simulink model "tractor_mu"  (R2022b)
settings: Solver=FixedStepDiscrete  StartTime=0.0  StopTime=20  FixedStep=0.001  RelTol=1e-3
model workspace (MAT data in the model file):
  P : object (value not decoded)
  w_2 : Simulink.Parameter (value not decoded)
undefined symbols (not defined in the file): A, a, B, b, C, D, DiscIntNeverNeededParam, Iz, K, k1, K1, k2, K2, L1, L2, m, magnitude, Phi, Sample_time, Steer_Ratio
libraries: simulink x26, slpidlib x13, Solver_SF x1, dsparch4 x1
(part 3 of 7)

== system tractor_mu/Dugoff轮胎模型/pac2002 ==
  lamda_fl : Inport
  lamda_fr : Inport  Port=2
  lamda_rl : Inport  Port=3
  lamda_rr : Inport  Port=4
  alpha_fl : Inport  Port=5
  alpha_fr : Inport  Port=6
  alpha_rl : Inport  Port=7
  alpha_rr : Inport  Port=8
  Fz_fl : Inport  Port=9
  Fz_rl : Inport  Port=10
  Fz_fr : Inport  Port=11
  Fz_rr : Inport  Port=12
  mu : Inport  Port=13
  Demux : Demux
  Gain{8..11} (4 alike) : Gain  Gain=-1
  fl_dugoff : MATLAB Function  TreatAsAtomicUnit=on
  fr_dugoff : MATLAB Function  TreatAsAtomicUnit=on
  rl_dugoff : MATLAB Function  TreatAsAtomicUnit=on
  rr_dugoff : MATLAB Function  TreatAsAtomicUnit=on
  Fx_fl : Outport
  Fx_fr : Outport  Port=2
  Fx_rl : Outport  Port=3
  Fx_rr : Outport  Port=4
  Fy_fl : Outport  Port=5
  Fy_fr : Outport  Port=6
  Fy_rl : Outport  Port=7
  Fy_rr : Outport  Port=8
  wires:
  alpha_fl/1 -> fl_dugoff/4(alpha)
  Fz_fl/1 -> fl_dugoff/1(Fz)
  alpha_rr/1 -> rr_dugoff/4(alpha)
  Fz_rr/1 -> rr_dugoff/1(Fz)
  [u_fl] -> fl_dugoff/2(u)
  [u_fr] -> fr_dugoff/2(u)
  alpha_fr/1 -> fr_dugoff/4(alpha)
  [u_rl] -> rl_dugoff/2(u)
  [u_rr] -> rr_dugoff/2(u)
  lamda_fr/1 -> Gain11/1
  lamda_rl/1 -> Gain8/1
  lamda_rr/1 -> Gain9/1
  lamda_fl/1 -> Gain10/1
  alpha_rl/1 -> rl_dugoff/4(alpha)
  Gain8/1 -> rl_dugoff/3(lamda)
  Gain9/1 -> rr_dugoff/3(lamda)
  Gain10/1 -> fl_dugoff/3(lamda)
  Gain11/1 -> fr_dugoff/3(lamda)
  mu/1 -> Demux/1
  Demux/1 -> [u_fl]
  Demux/2 -> [u_fr]
  Demux/3 -> [u_rl]
  Demux/4 -> [u_rr]
  Fz_rl/1 -> rl_dugoff/1(Fz)
  Fz_fr/1 -> fr_dugoff/1(Fz)
  fl_dugoff/4(Fy) -> Fy_fl/1
  fl_dugoff/3(Fx) -> Fx_fl/1
  fr_dugoff/4(Fy) -> Fy_fr/1
  fr_dugoff/3(Fx) -> Fx_fr/1
  rl_dugoff/4(Fy) -> Fy_rl/1
  rl_dugoff/3(Fx) -> Fx_rl/1
  rr_dugoff/4(Fy) -> Fy_rr/1
  rr_dugoff/3(Fx) -> Fx_rr/1

== system tractor_mu/PID_Controller//直线循迹/Enabled Subsystem ==
  note: DOB:仿真步长Ts=0.001，时间常数Tao=0.1
      | 如需部署到实车需要根据实车采样频率调整
  yaw_ref : Inport
  yaw : Inport  Port=2
  beta : Inport  Port=3
  omega : Inport  Port=4
  Enable : EnablePort  StatesWhenEnabling=reset
  5500/3000 : slpidlib/PID Controller  Controller=PID  Form=Parallel  TimeDomain=Discrete-time  UseExternalTs=off  SampleTime=-1  IntegratorMethod=Forward Euler  FilterMethod=Forward Euler  ControllerParametersSource=internal  P=5500  I=3500  UseKiTs=off  D=0  N=100  UseFilter=on  TunerSelectOption=Transfer Function Based (PID Tuner App)  InitialConditionSource=internal  InitialConditionForIntegrator=0  InitialConditionForFilter=0  DifferentiatorICPrevScaledInput=0  ExternalReset=none  TrackingMode=off  Kt=1  LimitOutput=off  SatLimitsSource=internal  UpperSaturationLimit=inf  LowerSaturationLimit=-inf  LinearizeAsGain=on  AntiWindupMode=none  Kb=1  LimitIntegrator=off  UpperIntegratorSaturationLimit=inf  LowerIntegratorSaturationLimit=-inf  POutMin=[]  POutMax=[]  IOutMin=[]  IOutMax=[]  DOutMin=[]  DOutMax=[]  NOutMin=[]  NOutMax=[]  SumOutMin=[]  SumOutMax=[]  SaturationOutMin=[]  SaturationOutMax=[]  PParamMin=[]  PParamMax=[]  IParamMin=[]  IParamMax=[]  DParamMin=[]  DParamMax=[]  NParamMin=[]  NParamMax=[]  KbParamMin=[]  KbParamMax=[]  KtParamMin=[]  KtParamMax=[]  KbOutMin=[]  KbOutMax=[]  KtOutMin=[]  KtOutMax=[]  IntegratorOutMin=[]  IntegratorOutMax=[]  FilterOutMin=[]  FilterOutMax=[]  SumI1OutMin=[]  SumI1OutMax=[]  SumI2OutMin=[]  SumI2OutMax=[]  SumI3OutMin=[]  SumI3OutMax=[]  SumI4OutMin=[]  SumI4OutMax=[]  SumDOutMin=[]  SumDOutMax=[]  DifferentiatorOutMin=[]  DifferentiatorOutMax=[]  FilterDiffOutCoefMin=[]  FilterDiffOutCoefMax=[]  ReciprocalOutMin=[]  ReciprocalOutMax=[]  SumDenOutMin=[]  SumDenOutMax=[]  SumNumOutMin=[]  SumNumOutMax=[]  DivideOutMin=[]  DivideOutMax=[]  UdiffTsProdOutMin=[]  UdiffTsProdOutMax=[]  NTsProdOutMin=[]  NTsProdOutMax=[]  UintegralTsProdOutMin=[]  UintegralTsProdOutMax=[]  UngainTsProdOutMin=[]  UngainTsProdOutMax=[]  ClampingZeroOutDataTypeStr=Inherit: Inherit via back propagation  ClampingZeroOutMin=[]  ClampingZeroOutMax=[]  FilterDenConstantOutDataTypeStr=Inherit: Inherit via back propagation  FilterDenConstantOutMin=[]  FilterDenConstantOutMax=[]  PCopyOutDataTypeStr=Inherit: Inherit via back propagation  PCopyOutMin=[]  PCopyOutMax=[]  NCopyOutDataTypeStr=Inherit: Inherit via back propagation  NCopyOutMin=[]  NCopyOutMax=[]  IntegratorContinuousStateAttributes=''  IntegratorStateMustResolveToSignalObject=off  IntegratorRTWStateStorageClass=Auto  FilterContinuousStateAttributes=''  FilterStateMustResolveToSignalObject=off  FilterRTWStateStorageClass=Auto  ParallelPVariant=InternalParameters  IdealPVariant=Disabled  IVariant=InternalParameters  DVariant=InternalParameters  IntegratorVariant=Discrete  SatVariant=Disabled  AWVariant=Passthrough  PCopyVariant=Disabled  TRVariant=Disabled  FdbkBlocksVariant=Forward  IdealPFdbkVariant=Disabled  SatFdbkVariant=Disabled  DerivativeFilterVariant=ForwardEulerFilter  NVariant=InternalParameters  NCopyVariant=Disabled  FilterICVariant=InternalICsFilter  IntegratorICVariant=InternalICs  ExternalResetVariant=Disabled  TRSumVariant=Passthrough  SumFdbkVariant=Disabled  SumVariant=Sum_PID  TsampFilterVariant=InternalTs  TsampNgainVariant=Passthrough  TsampIntegralVariant=Passthrough  ExternalSaturationOutDataTypeStr=Inherit: Same as second input
  Add : Sum  Inputs=+++
  Data Type Conversion : DataTypeConversion  OutDataTypeStr=single  SaturateOnIntegerOverflow=off  RndMeth=Floor
  Data Type Conversion1 : DataTypeConversion  OutDataTypeStr=single  SaturateOnIntegerOverflow=off  RndMeth=Floor
  Discrete Transfer Fcn : DiscreteTransferFcn  Numerator=[1-exp(-0.2)]  Denominator=[1 -exp(-0.2)]
  Gain : Gain  Gain=-1
  Gain1 : Gain  Gain=-K(1)
  Gain2 : Gain  Gain=-K(2)
  Gain3 : Gain  Gain=-K(3)
  Gain4 : Gain  Gain=3
  Gain5 : Gain  Gain=0.5
  Gain6 : Gain  Gain=180/pi
  Izr_dot : simulink/Discrete/Discrete Derivative  gainval=67536  ICPrevScaledInput=0.0  OutMin=[]  OutMax=[]  OutDataType=fixdt(1, 16)  OutScaling=2^-10  DoSatur=off
  Manual Switch : ManualSwitch
  Manual Switch1 : ManualSwitch
  Subtract : Sum  Inputs=+-
  Sum : Sum  Inputs=|+-
  Sum2 : Sum  Inputs=|+-
  Mz : Outport
  wires:
  5500/3000/1 -> Data Type Conversion1/1
  yaw_ref/1 -> Sum/1
  yaw/1 -> Sum/2
  Sum/1 -> Gain/1, Gain6/1
  Sum2/1 -> Manual Switch/2
  Discrete Transfer Fcn/1 -> Gain5/1
  Subtract/1 -> Discrete Transfer Fcn/1
  Gain3/1 -> Add/3  "eyaw"
  Gain1/1 -> Add/1  "beta"
  Izr_dot/1 -> Subtract/1
  omega/1 -> Izr_dot/1, Gain2/1
  Gain2/1 -> Add/2  "omega"
  Add/1 -> Gain4/1
  beta/1 -> Gain1/1
  Gain/1 -> Gain3/1
  Manual Switch/1 -> Manual Switch1/2
  Manual Switch1/1 -> Mz/1
  Gain4/1 -> Subtract/2, Manual Switch/1, Sum2/1
  Data Type Conversion/1 -> Sum2/2  "Mz_DOB"
  Data Type Conversion1/1 -> Manual Switch1/1  "Mz_pid"
  Gain5/1 -> Data Type Conversion/1
  Gain6/1 -> 5500/3000/1

== system tractor_mu/PID_Controller//直线循迹/目标航向角计算 ==
  reset : Inport
  yaw : Inport  Port=2
  omega : Inport  Port=3
  Enable : EnablePort  StatesWhenEnabling=reset
  Abs : Abs  SaturateOnIntegerOverflow=off
  Add : Sum
  Constant : Constant
  Constant1 : Constant  Value=0.001
  Discrete-Time Integrator : DiscreteIntegrator  ExternalReset=rising  SampleTime=-1  ICPrevOutput=DiscIntNeverNeededParam  ICPrevScaledInput=DiscIntNeverNeededParam
  Discrete-Time Integrator1 : DiscreteIntegrator  ExternalReset=rising  SampleTime=-1  ICPrevOutput=DiscIntNeverNeededParam  ICPrevScaledInput=DiscIntNeverNeededParam
  Divide : Product  Inputs=*/
  Divide1 : Product  Inputs=*/
  Product : Product
  Saturation : Saturate  UpperLimit=999999  LowerLimit=0.1
  yaw_r : Outport
  wires:
  Constant/1 -> Divide/1
  omega/1 -> Abs/1
  Abs/1 -> Add/1
  Constant1/1 -> Add/2
  Add/1 -> Divide/2
  Divide/1 -> Discrete-Time Integrator1/1, Product/2
  yaw/1 -> Product/1
  Product/1 -> Discrete-Time Integrator/1
  Discrete-Time Integrator/1 -> Divide1/1
  Discrete-Time Integrator1/1 -> Saturation/1
  Divide1/1 -> yaw_r/1
  Saturation/1 -> Divide1/2
  reset/1 -> Discrete-Time Integrator1/2, Discrete-Time Integrator/2

== system tractor_mu/协同博弈扭矩分配/Subsystem ==
  Tflref : Inport
  Tfrref : Inport  Port=2
  Trlref : Inport  Port=3
  Trrref : Inport  Port=4
  Tflbase : Inport  Port=5
  Tfrbase : Inport  Port=6
  Trlbase : Inport  Port=7
  Trrbase : Inport  Port=8
  alpha : Inport  Port=9
  Constant{,1..3} (4 alike) : Constant
  Product{,1..7} (8 alike) : Product
  Sum{,2,4,6} (4 alike) : Sum  Inputs=|+-
  Sum{1,3,5,7} (4 alike) : Sum  Inputs=|++
  alpha1 : InportShadow  Port=9
  alpha2 : InportShadow  Port=9
  alpha3 : InportShadow  Port=9
  Tfl_sh : Outport
  Tfr_sh : Outport  Port=2
  Trl_sh : Outport  Port=3
  Trr_sh : Outport  Port=4
  wires:
  Tflbase/1 -> Product/1
  Constant/1 -> Sum/1
  alpha/1 -> Sum/2, Product1/2
  Sum/1 -> Product/2
  Product/1 -> Sum1/1
  Product1/1 -> Sum1/2
  Tflref/1 -> Product1/1
  Sum1/1 -> Tfl_sh/1
  Sum3/1 -> Tfr_sh/1
  Tfrref/1 -> Product3/1
  Product3/1 -> Sum3/2
  Product2/1 -> Sum3/1
  Sum2/1 -> Product2/2
  alpha1/1 -> Product3/2, Sum2/2
  Constant1/1 -> Sum2/1
  Tfrbase/1 -> Product2/1
  Trlbase/1 -> Product4/1
  Constant2/1 -> Sum4/1
  alpha2/1 -> Sum4/2, Product5/2
  Sum4/1 -> Product4/2
  Product4/1 -> Sum5/1
  Product5/1 -> Sum5/2
  Trlref/1 -> Product5/1
  Sum5/1 -> Trl_sh/1
  Sum7/1 -> Trr_sh/1
  Trrref/1 -> Product7/1
  Product7/1 -> Sum7/2
  Product6/1 -> Sum7/1
  Sum6/1 -> Product6/2
  alpha3/1 -> Product7/2, Sum6/2
  Constant3/1 -> Sum6/1
  Trrbase/1 -> Product6/1

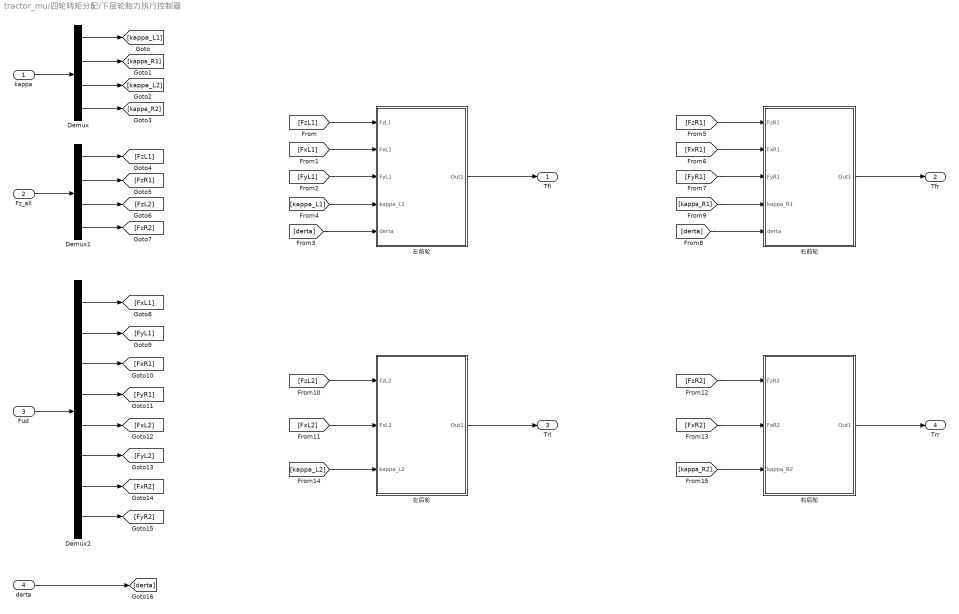
== system tractor_mu/四轮转矩分配/下层轮胎力执行控制器 ==
  kappa : Inport
  Fz_all : Inport  Port=2
  Fud : Inport  Port=3
  derta : Inport  Port=4
  Demux : Demux
  Demux1 : Demux
  Demux2 : Demux  Outputs=8
  右前轮 : Subsystem
  右后轮 : Subsystem
  左前轮 : Subsystem
  左后轮 : Subsystem
  Tfl : Outport
  Tfr : Outport  Port=2
  Trl : Outport  Port=3
  Trr : Outport  Port=4
  wires:
  kappa/1 -> Demux/1
  Demux/1 -> [kappa_L1]
  Demux/2 -> [kappa_R1]
  Demux/3 -> [kappa_L2]
  Demux/4 -> [kappa_R2]
  Fz_all/1 -> Demux1/1
  Demux1/1 -> [FzL1]
  Demux1/2 -> [FzR1]
  Demux1/3 -> [FzL2]
  Demux1/4 -> [FzR2]
  Fud/1 -> Demux2/1
  Demux2/1 -> [FxL1]
  Demux2/2 -> [FyL1]
  Demux2/3 -> [FxR1]
  Demux2/4 -> [FyR1]
  Demux2/6 -> [FyL2]
  Demux2/5 -> [FxL2]
  Demux2/8 -> [FyR2]
  Demux2/7 -> [FxR2]
  derta/1 -> [derta]
  左前轮/1(Out1) -> Tfl/1
  [FzL1] -> 左前轮/1(FzL1)
  [FxL1] -> 左前轮/2(FxL1)
  [FyL1] -> 左前轮/3(FyL1)
  [kappa_L1] -> 左前轮/4(kappa_L1)
  [derta] -> 左前轮/5(derta)
  [derta] -> 右前轮/5(derta)
  [kappa_R1] -> 右前轮/4(kappa_R1)
  [FyR1] -> 右前轮/3(FyR1)
  [FxR1] -> 右前轮/2(FxR1)
  [FzR1] -> 右前轮/1(FzR1)
  右前轮/1(Out1) -> Tfr/1
  [kappa_L2] -> 左后轮/3(kappa_L2)
  [FxL2] -> 左后轮/2(FxL2)
  [FzL2] -> 左后轮/1(FzL2)
  左后轮/1(Out1) -> Trl/1
  右后轮/1(Out1) -> Trr/1
  [FzR2] -> 右后轮/1(FzR2)
  [FxR2] -> 右后轮/2(FxR2)
  [kappa_R2] -> 右后轮/3(kappa_R2)

== system tractor_mu/总驱动力矩制定/DOB补偿 ==
  note: 仿真时间t=0.001
      | 时间常数tao=0.1
  vx : Inport
  T : Inport  Port=2
  Discrete Transfer Fcn : DiscreteTransferFcn  Numerator=[1 1]  Denominator=[201 -199]
  Discrete Derivative : simulink/Discrete/Discrete Derivative  gainval=1.0  ICPrevScaledInput=0.0  OutMin=[]  OutMax=[]  OutDataType=fixdt(1, 16)  OutScaling=2^-10  DoSatur=off
  Sum : Sum  Inputs=|-+
  m*Rf : Gain  Gain=18530*0.834
  低通LPF : DiscreteTransferFcn  Numerator=[1-0.9802]  Denominator=[1 -0.9802]
  Td_hat : Outport
  wires:
  Discrete Derivative/1 -> m*Rf/1
  vx/1 -> 低通LPF/1
  m*Rf/1 -> Sum/1
  T/1 -> Sum/2
  Sum/1 -> Discrete Transfer Fcn/1
  Discrete Transfer Fcn/1 -> Td_hat/1
  低通LPF/1 -> Discrete Derivative/1

== system tractor_mu/总驱动力矩制定/正常工况_高速衰减防抖 ==
  gearD : Inport
  vx : Inport  Port=2
  T0 : Inport  Port=3
  1档 : Switch  Criteria=u2 > Threshold  Threshold=14/3.6  SaturateOnIntegerOverflow=off  InputSameDT=off
  2档 : Switch  Criteria=u2 > Threshold  Threshold=40  SaturateOnIntegerOverflow=off  InputSameDT=off
  Gain14 : Gain  Gain=3.6
  Subsystem1 : Subsystem
  Switch5 : Switch  Criteria=u2 > Threshold  Threshold=1  SaturateOnIntegerOverflow=off  InputSameDT=off
  高速衰减冻结区 : Subsystem
  T : Outport
  wires:
  vx/1 -> 1档/2, Gain14/1
  Gain14/1 -> Subsystem1/1(v), 2档/2, 高速衰减冻结区/1(v)
  T0/1 -> 2档/3, 1档/3
  1档/1 -> Switch5/3
  Subsystem1/1(Out1) -> 2档/1
  高速衰减冻结区/1(Out1) -> 1档/1
  gearD/1 -> Switch5/2
  2档/1 -> Switch5/1
  Switch5/1 -> T/1

== system tractor_mu/牵引效率计算/Subsystem1 ==
  T : Inport
  F_hat : Inport  Port=2
  wij : Inport  Port=3
  Fz : Inport  Port=4
  Add : Sum  Inputs=+++-
  Gain : Gain  Gain=50
  Jw : Gain  Gain=1/356.42
  Product : Product
  Saturation : Saturate  UpperLimit=1  LowerLimit=-1
  Sum : Sum  Inputs=|+-
  边界层厚度 : Gain  Gain=1/1
  Fx_out : Outport
  wires:
  wij/1 -> Sum/1
  Sum/1 -> Gain/1, 边界层厚度/1
  边界层厚度/1 -> Saturation/1
  Saturation/1 -> Product/2  "us"
  T/1 -> Jw/1
  Jw/1 -> Add/1
  Gain/1 -> Add/2
  Product/1 -> Add/3

== system tractor_mu/牵引效率计算/总纵向力估计 ==
  ax : Inport
  theta : Inport  Port=2
  EFsum : Inport  Port=3
  vx : Inport  Port=4
  Fz4 : Inport  Port=5
  Add : Sum  Inputs=---+
  Add1 : Sum  Inputs=++++
  Delay : Delay  DelayLength=1
  Demux : Demux
  Gain1 : Gain  Gain=2.4516
  Gain3 : Gain  Gain=18530*9.8
  Gain5 : Gain  Gain=18530
  Math Function : Math  Operator=magnitude^2
  Saturation : Saturate  UpperLimit=999999999  LowerLimit=0
  Saturation1 : Saturate  UpperLimit=999999999  LowerLimit=0
  Saturation2 : Saturate  UpperLimit=999999999  LowerLimit=0
  Sin1 : Trigonometry
  Sum : Sum  Inputs=|+-
  Switch : Switch  Criteria=u2 > Threshold  Threshold=0.5  SaturateOnIntegerOverflow=off  InputSameDT=off
  滚动阻力系数 : Gain  Gain=0.02
  R_load : Outport
  R_all : Outport  Port=2
  R_g : Outport  Port=3
  R_f : Outport  Port=4
  R_a : Outport  Port=5
  wires:
  ax/1 -> Gain5/1
  theta/1 -> Sin1/1
  Gain1/1 -> R_a/1, Add/2
  Sin1/1 -> Gain3/1
  Gain3/1 -> R_g/1, Add/3
  Add/1 -> Saturation/1
  EFsum/1 -> Sum/1
  Gain5/1 -> Sum/2
  Sum/1 -> Delay/1, Add/4, Saturation1/1
  Fz4/1 -> Demux/1
  Demux/1 -> Add1/1
  Demux/2 -> Add1/2
  Demux/3 -> Add1/3
  Demux/4 -> Add1/4
  Add1/1 -> 滚动阻力系数/1
  滚动阻力系数/1 -> Add/1, R_f/1
  vx/1 -> Switch/2, Math Function/1
  Math Function/1 -> Gain1/1
  Saturation/1 -> R_load/1
  Saturation1/1 -> Switch/1
  Switch/1 -> R_all/1
  Delay/1 -> Saturation2/1
  Saturation2/1 -> Switch/3

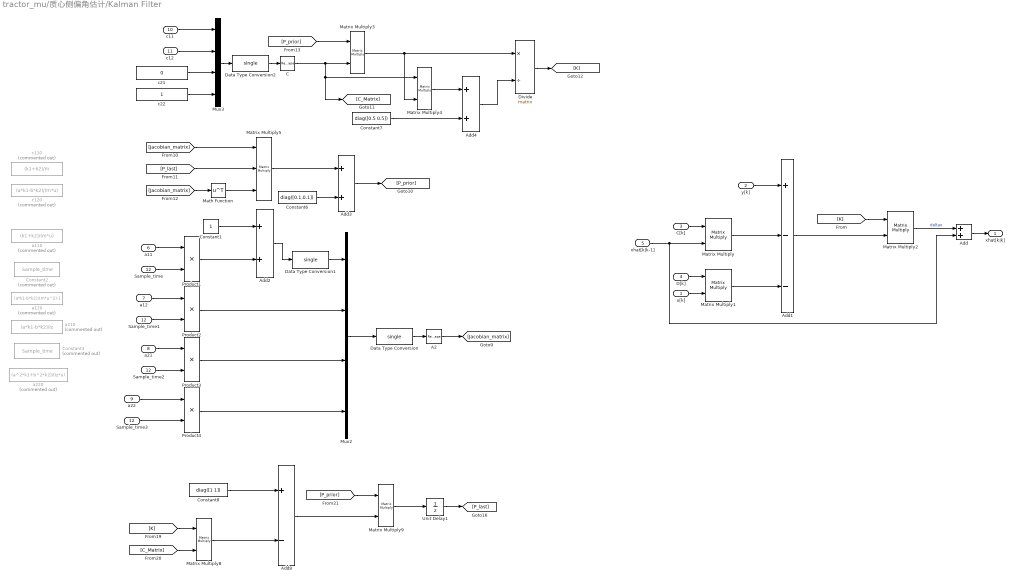
== system tractor_mu/质心侧偏角估计/Kalman Filter ==
  u[k] : Inport
  y[k] : Inport  Port=2
  C[k] : Inport  Port=3
  D[k] : Inport  Port=4
  xhat[k|k-1] : Inport  Port=5
  a11 : Inport  Port=6  OutDataTypeStr=single
  a12 : Inport  Port=7  OutDataTypeStr=single
  a21 : Inport  Port=8  OutDataTypeStr=single
  a22 : Inport  Port=9  OutDataTypeStr=single
  c11 : Inport  Port=10  OutDataTypeStr=single
  c12 : Inport  Port=11  OutDataTypeStr=single
  Sample_time : Inport  Port=12  OutDataTypeStr=single
  A2 : Reshape  OutputDimensionality=Customize  OutputDimensions=[2,2]
  Add{,2..4} (4 alike) : Sum
  Add1 : Sum  Inputs=+--
  Add8 : Sum  Inputs=+-
  C : Reshape  OutputDimensionality=Customize  OutputDimensions=[2,2]
  Constant1 : Constant
  Constant2 : Constant  Commented=on  Value=Sample_time
  Constant3 : Constant  Commented=on  Value=Sample_time
  Constant6 : Constant  Value=diag([0.1,0.1])
  Constant7 : Constant  Value=diag([0.5 0.5])
  Constant8 : Constant  Value=diag([1 1])
  Data Type Conversion : DataTypeConversion  OutDataTypeStr=single  SaturateOnIntegerOverflow=off  RndMeth=Floor
  Data Type Conversion1 : DataTypeConversion  OutDataTypeStr=single  SaturateOnIntegerOverflow=off  RndMeth=Floor
  Data Type Conversion2 : DataTypeConversion  OutDataTypeStr=single  SaturateOnIntegerOverflow=off  RndMeth=Floor
  Divide : Product  Inputs=*/  Multiplication=Matrix(*)
  Math Function : Math  Operator=transpose  SignedPower=on
  Matrix Multiply{,1..4,8..9} (7 alike) : Product  Multiplication=Matrix(*)
  Matrix Multiply5 : Product  Inputs=3  Multiplication=Matrix(*)
  Mux2 : Mux
  Mux3 : Mux
  Product1 : Product
  Product2 : Product
  Product3 : Product  OutDataTypeStr=single
  Product4 : Product  OutDataTypeStr=single
  Sample_time1 : InportShadow  Port=12  OutDataTypeStr=single
  Sample_time2 : InportShadow  Port=12  OutDataTypeStr=single
  Sample_time3 : InportShadow  Port=12  OutDataTypeStr=single
  Unit Delay1 : UnitDelay  SampleTime=-1  HasFrameUpgradeWarning=on
  a110 : Constant  Commented=on  Value=(k1+k2)/(m*u)
  a120 : Constant  Commented=on  Value=(a*k1-b*k2)/(m*u^2)-1
  a210 : Constant  Commented=on  Value=(a*k1-b*k2)/Iz
  a220 : Constant  Commented=on  Value=(a^2*k1+b^2*k2)/(Iz*u)
  c110 : Constant  Commented=on  Value=(k1+k2)/m
  c120 : Constant  Commented=on  Value=(a*k1-b*k2)/(m*u)
  c21 : Constant  Value=0  OutDataTypeStr=single
  c22 : Constant  OutDataTypeStr=single
  xhat[k|k] : Outport
  wires:
  Add/1 -> xhat[k|k]/1
  C[k]/1 -> Matrix Multiply/1
  xhat[k|k-1]/1 -> Matrix Multiply/2, Add/2
  D[k]/1 -> Matrix Multiply1/1
  u[k]/1 -> Matrix Multiply1/2
  y[k]/1 -> Add1/1
  Matrix Multiply/1 -> Add1/2
  Matrix Multiply1/1 -> Add1/3
  Add1/1 -> Matrix Multiply2/2
  Matrix Multiply2/1 -> Add/1  "deltax"
  Add4/1 -> Divide/2
  Matrix Multiply3/1 -> Divide/1, Matrix Multiply4/2
  c21/1 -> Mux3/3
  Matrix Multiply4/1 -> Add4/1
  c22/1 -> Mux3/4
  Mux3/1 -> Data Type Conversion2/1
  Constant7/1 -> Add4/2
  c11/1 -> Mux3/1
  [P_prior] -> Matrix Multiply3/1
  C/1 -> Matrix Multiply4/1, [C_Matrix], Matrix Multiply3/2
  Divide/1 -> [K]
  [P_last] -> Matrix Multiply5/2
  Matrix Multiply5/1 -> Add3/1
  [Jacobian_matrix] -> Math Function/1
  Math Function/1 -> Matrix Multiply5/3
  Add3/1 -> [P_prior]
  [Jacobian_matrix] -> Matrix Multiply5/1
  Constant6/1 -> Add3/2
  Sample_time2/1 -> Product3/2
  Sample_time3/1 -> Product4/2
  a12/1 -> Product2/1
  A2/1 -> [Jacobian_matrix]
  Add2/1 -> Data Type Conversion1/1
  Product1/1 -> Add2/2
  Sample_time1/1 -> Product2/2
  a22/1 -> Product4/1
  Mux2/1 -> Data Type Conversion/1
  a21/1 -> Product3/1
  Constant1/1 -> Add2/1
  [K] -> Matrix Multiply2/1
  Matrix Multiply8/1 -> Add8/2
  Constant8/1 -> Add8/1
  Unit Delay1/1 -> [P_last]
  [P_prior] -> Matrix Multiply9/1
  Add8/1 -> Matrix Multiply9/2
  Matrix Multiply9/1 -> Unit Delay1/1
  [K] -> Matrix Multiply8/1
  [C_Matrix] -> Matrix Multiply8/2
  a11/1 -> Product1/1
  c12/1 -> Mux3/2
  Sample_time/1 -> Product1/2
  Product2/1 -> Mux2/2
  Product3/1 -> Mux2/3
  Product4/1 -> Mux2/4
  Data Type Conversion/1 -> A2/1
  Data Type Conversion1/1 -> Mux2/1
  Data Type Conversion2/1 -> C/1

== system tractor_mu/质心侧偏角估计/Observer ==
  note: A*xhat+B*u+L*(yMeas-yHat)
      | or
      | A*xhat+B*u
  u[k] : Inport
  y[k] : Inport  Port=2
  A[k] : Inport  Port=3
  B[k] : Inport  Port=4
  C[k] : Inport  Port=5
  D[k] : Inport  Port=6
  L[k] : Inport  Port=7
  xhat[k|k-1] : Inport  Port=8
  Add : Sum  Inputs=+++
  Matrix Multiply : Product  Multiplication=Matrix(*)
  Matrix Multiply1 : Product  Multiplication=Matrix(*)
  Reshape : Reshape
  Subsystem : Subsystem
  x[k+1|k] : Outport
  wires:
  B[k]/1 -> Matrix Multiply/1
  u[k]/1 -> Subsystem/6(u[k]), Matrix Multiply/2
  A[k]/1 -> Matrix Multiply1/1
  xhat[k|k-1]/1 -> Matrix Multiply1/2, Subsystem/4(xhat[k|k-1])
  L[k]/1 -> Subsystem/1(L[k])
  y[k]/1 -> Subsystem/2(y[k])
  C[k]/1 -> Subsystem/3(C[k])
  D[k]/1 -> Subsystem/5(D[k])
  Matrix Multiply/1 -> Add/1
  Matrix Multiply1/1 -> Add/2
  Subsystem/1(L*(y[k]-yhat[k|k-1])) -> Add/3
  Add/1 -> Reshape/1
  Reshape/1 -> x[k+1|k]/1

== system tractor_mu/质心侧偏角滑模观测器估计/Subsystem ==
  Avz_Carsim : Inport
  vx : Inport  Port=2
  delta_f : Inport  Port=3
  Atan : Trigonometry  Operator=atan
  Constant : Constant  Value=0.1
  Divide : Product  Inputs=*/
  Gain1 : Gain  Gain=L1
  Gain2 : Gain  Gain=L2
  MATLAB Function : MATLAB Function  TreatAsAtomicUnit=on  SystemSampleTime=0.005
  Scope1 : Scope
  Scope2 : Scope
  Subsystem : Subsystem
  Sum : Sum  Inputs=|+-
  Sum1 : Sum  Inputs=|++
  Sum2 : Sum  Inputs=|++
  Switch : Switch  Criteria=u2 > Threshold  Threshold=0.1  SaturateOnIntegerOverflow=off  InputSameDT=off
  gamma_hat : DiscreteIntegrator  SampleTime=-1  ICPrevOutput=DiscIntNeverNeededParam  ICPrevScaledInput=DiscIntNeverNeededParam
  vy_hat : DiscreteIntegrator  SampleTime=-1  ICPrevOutput=DiscIntNeverNeededParam  ICPrevScaledInput=DiscIntNeverNeededParam
  beta_est : Outport
  gamma_est : Outport  Port=2
  vy_hat_output : Outport  Port=3
  wires:
  Avz_Carsim/1 -> Sum/1
  Sum/1 -> Subsystem/1(error)
  MATLAB Function/1(d_vy_model) -> Sum1/2
  gamma_hat/1 -> Scope1/1, MATLAB Function/4(gamma_hat), gamma_est/1, Sum/2
  vx/1 -> Scope2/1, Switch/1, Switch/2
  Constant/1 -> Switch/3
  vy_hat/1 -> vy_hat_output/1, Divide/1, MATLAB Function/3(vy_hat)
  Switch/1 -> Divide/2, MATLAB Function/1(vx)
  Subsystem/1(v_STA) -> Gain2/1, Gain1/1
  delta_f/1 -> MATLAB Function/2(delta_f)
  Divide/1 -> Atan/1
  Gain1/1 -> Sum1/1
  Gain2/1 -> Sum2/1
  MATLAB Function/2(d_gamma_model) -> Sum2/2
  Atan/1 -> beta_est/1
  Sum1/1 -> vy_hat/1
  Sum2/1 -> gamma_hat/1

== system tractor_mu/质心侧偏角滑模观测器估计/Subsystem1 ==
  Avz_Carsim : Inport
  vx : Inport  Port=2
  delta_f : Inport  Port=3
  Atan : Trigonometry  Operator=atan
  Constant : Constant  Value=0.1
  Divide : Product  Inputs=*/
  Gain : Gain  Gain=1/Phi
  Gain1 : Gain  Gain=L1
  Gain2 : Gain  Gain=L2
  MATLAB Function : MATLAB Function  TreatAsAtomicUnit=on  SystemSampleTime=0.005
  Saturation : Saturate  UpperLimit=1  LowerLimit=-1
  Scope1 : Scope
  Scope2 : Scope
  Sum : Sum  Inputs=|+-
  Sum1 : Sum  Inputs=|++
  Sum2 : Sum  Inputs=|++
  Switch : Switch  Criteria=u2 > Threshold  Threshold=0.1  SaturateOnIntegerOverflow=off  InputSameDT=off
  gamma_hat : Integrator
  vy_hat : Integrator
  beta_est : Outport
  gamma_est : Outport  Port=2
  vy_hat_output : Outport  Port=3
  wires:
  Gain/1 -> Saturation/1
  Avz_Carsim/1 -> Sum/1
  Sum/1 -> Gain/1
  MATLAB Function/1(d_vy_model) -> Sum1/2
  gamma_hat/1 -> Scope1/1, MATLAB Function/4(gamma_hat), gamma_est/1, Sum/2
  vx/1 -> Scope2/1, Switch/1, Switch/2
  Constant/1 -> Switch/3
  vy_hat/1 -> vy_hat_output/1, Divide/1, MATLAB Function/3(vy_hat)
  Switch/1 -> Divide/2, MATLAB Function/1(vx)
  Saturation/1 -> Gain2/1, Gain1/1
  delta_f/1 -> MATLAB Function/2(delta_f)
  Divide/1 -> Atan/1
  Gain1/1 -> Sum1/1
  Gain2/1 -> Sum2/1
  MATLAB Function/2(d_gamma_model) -> Sum2/2
  Atan/1 -> beta_est/1
  Sum1/1 -> vy_hat/1
  Sum2/1 -> gamma_hat/1

== system tractor_mu/驱动防滑模块/Subsystem ==
  lamda1 : Inport
  p : Inport  Port=2
  i : Inport  Port=3
  b : Inport  Port=4
  Constant : Constant  Value=0.2
  PID Controller : slpidlib/PID Controller  Controller=PI  Form=Parallel  TimeDomain=Discrete-time  UseExternalTs=off  SampleTime=-1  IntegratorMethod=Forward Euler  FilterMethod=Forward Euler  ControllerParametersSource=external  P=5000  I=3000  UseKiTs=off  D=0  N=100  UseFilter=on  TunerSelectOption=Transfer Function Based (PID Tuner App)  InitialConditionSource=internal  InitialConditionForIntegrator=0  InitialConditionForFilter=0  DifferentiatorICPrevScaledInput=0  ExternalReset=none  TrackingMode=off  Kt=1  LimitOutput=on  SatLimitsSource=internal  UpperSaturationLimit=0  LowerSaturationLimit=-30000  LinearizeAsGain=on  AntiWindupMode=clamping  Kb=1  LimitIntegrator=off  UpperIntegratorSaturationLimit=inf  LowerIntegratorSaturationLimit=-inf  POutMin=[]  POutMax=[]  IOutMin=[]  IOutMax=[]  DOutMin=[]  DOutMax=[]  NOutMin=[]  NOutMax=[]  SumOutMin=[]  SumOutMax=[]  SaturationOutMin=[]  SaturationOutMax=[]  PParamMin=[]  PParamMax=[]  IParamMin=[]  IParamMax=[]  DParamMin=[]  DParamMax=[]  NParamMin=[]  NParamMax=[]  KbParamMin=[]  KbParamMax=[]  KtParamMin=[]  KtParamMax=[]  KbOutMin=[]  KbOutMax=[]  KtOutMin=[]  KtOutMax=[]  IntegratorOutMin=[]  IntegratorOutMax=[]  FilterOutMin=[]  FilterOutMax=[]  SumI1OutMin=[]  SumI1OutMax=[]  SumI2OutMin=[]  SumI2OutMax=[]  SumI3OutMin=[]  SumI3OutMax=[]  SumI4OutMin=[]  SumI4OutMax=[]  SumDOutMin=[]  SumDOutMax=[]  DifferentiatorOutMin=[]  DifferentiatorOutMax=[]  FilterDiffOutCoefMin=[]  FilterDiffOutCoefMax=[]  ReciprocalOutMin=[]  ReciprocalOutMax=[]  SumDenOutMin=[]  SumDenOutMax=[]  SumNumOutMin=[]  SumNumOutMax=[]  DivideOutMin=[]  DivideOutMax=[]  UdiffTsProdOutMin=[]  UdiffTsProdOutMax=[]  NTsProdOutMin=[]  NTsProdOutMax=[]  UintegralTsProdOutMin=[]  UintegralTsProdOutMax=[]  UngainTsProdOutMin=[]  UngainTsProdOutMax=[]  ClampingZeroOutDataTypeStr=Inherit: Inherit via back propagation  ClampingZeroOutMin=[]  ClampingZeroOutMax=[]  FilterDenConstantOutDataTypeStr=Inherit: Inherit via back propagation  FilterDenConstantOutMin=[]  FilterDenConstantOutMax=[]  PCopyOutDataTypeStr=Inherit: Inherit via back propagation  PCopyOutMin=[]  PCopyOutMax=[]  NCopyOutDataTypeStr=Inherit: Inherit via back propagation  NCopyOutMin=[]  NCopyOutMax=[]  IntegratorContinuousStateAttributes=''  IntegratorStateMustResolveToSignalObject=off  IntegratorRTWStateStorageClass=Auto  FilterContinuousStateAttributes=''  FilterStateMustResolveToSignalObject=off  FilterRTWStateStorageClass=Auto  ParallelPVariant=ExternalParameters  IdealPVariant=Disabled  IVariant=ExternalParameters  DVariant=Disabled  IntegratorVariant=Discrete  SatVariant=Enabled  AWVariant=DiscClampingParallel  PCopyVariant=Disabled  TRVariant=Disabled  FdbkBlocksVariant=Forward  IdealPFdbkVariant=Disabled  SatFdbkVariant=Disabled  DerivativeFilterVariant=Disabled  NVariant=Disabled  NCopyVariant=Disabled_SignalSpec  FilterICVariant=Disabled  IntegratorICVariant=InternalICs  ExternalResetVariant=Disabled  TRSumVariant=Passthrough  SumFdbkVariant=Disabled  SumVariant=Sum_PI  TsampFilterVariant=InternalTs  TsampNgainVariant=Passthrough  TsampIntegralVariant=Passthrough  ExternalSaturationOutDataTypeStr=Inherit: Same as second input
  Saturation : Saturate  UpperLimit=30000  LowerLimit=-30000
  Sum4 : Sum  Inputs=|+-
  dT1 : Outport
  wires:
  Sum4/1 -> PID Controller/1
  lamda1/1 -> Sum4/2
  PID Controller/1 -> Saturation/1  "dT1"
  p/1 -> PID Controller/2
  i/1 -> PID Controller/3
  Constant/1 -> Sum4/1
  Saturation/1 -> dT1/1

== system tractor_mu/驱动防滑模块/Subsystem1 ==
  lamda2 : Inport
  p : Inport  Port=2
  i : Inport  Port=3
  b : Inport  Port=4
  Constant : Constant  Value=0.2
  PID Controller : slpidlib/PID Controller  Controller=PI  Form=Parallel  TimeDomain=Discrete-time  UseExternalTs=off  SampleTime=-1  IntegratorMethod=Forward Euler  FilterMethod=Forward Euler  ControllerParametersSource=external  P=5000  I=3000  UseKiTs=off  D=0  N=100  UseFilter=on  TunerSelectOption=Transfer Function Based (PID Tuner App)  InitialConditionSource=internal  InitialConditionForIntegrator=0  InitialConditionForFilter=0  DifferentiatorICPrevScaledInput=0  ExternalReset=none  TrackingMode=off  Kt=1  LimitOutput=on  SatLimitsSource=internal  UpperSaturationLimit=0  LowerSaturationLimit=-30000  LinearizeAsGain=on  AntiWindupMode=clamping  Kb=1  LimitIntegrator=off  UpperIntegratorSaturationLimit=inf  LowerIntegratorSaturationLimit=-inf  POutMin=[]  POutMax=[]  IOutMin=[]  IOutMax=[]  DOutMin=[]  DOutMax=[]  NOutMin=[]  NOutMax=[]  SumOutMin=[]  SumOutMax=[]  SaturationOutMin=[]  SaturationOutMax=[]  PParamMin=[]  PParamMax=[]  IParamMin=[]  IParamMax=[]  DParamMin=[]  DParamMax=[]  NParamMin=[]  NParamMax=[]  KbParamMin=[]  KbParamMax=[]  KtParamMin=[]  KtParamMax=[]  KbOutMin=[]  KbOutMax=[]  KtOutMin=[]  KtOutMax=[]  IntegratorOutMin=[]  IntegratorOutMax=[]  FilterOutMin=[]  FilterOutMax=[]  SumI1OutMin=[]  SumI1OutMax=[]  SumI2OutMin=[]  SumI2OutMax=[]  SumI3OutMin=[]  SumI3OutMax=[]  SumI4OutMin=[]  SumI4OutMax=[]  SumDOutMin=[]  SumDOutMax=[]  DifferentiatorOutMin=[]  DifferentiatorOutMax=[]  FilterDiffOutCoefMin=[]  FilterDiffOutCoefMax=[]  ReciprocalOutMin=[]  ReciprocalOutMax=[]  SumDenOutMin=[]  SumDenOutMax=[]  SumNumOutMin=[]  SumNumOutMax=[]  DivideOutMin=[]  DivideOutMax=[]  UdiffTsProdOutMin=[]  UdiffTsProdOutMax=[]  NTsProdOutMin=[]  NTsProdOutMax=[]  UintegralTsProdOutMin=[]  UintegralTsProdOutMax=[]  UngainTsProdOutMin=[]  UngainTsProdOutMax=[]  ClampingZeroOutDataTypeStr=Inherit: Inherit via back propagation  ClampingZeroOutMin=[]  ClampingZeroOutMax=[]  FilterDenConstantOutDataTypeStr=Inherit: Inherit via back propagation  FilterDenConstantOutMin=[]  FilterDenConstantOutMax=[]  PCopyOutDataTypeStr=Inherit: Inherit via back propagation  PCopyOutMin=[]  PCopyOutMax=[]  NCopyOutDataTypeStr=Inherit: Inherit via back propagation  NCopyOutMin=[]  NCopyOutMax=[]  IntegratorContinuousStateAttributes=''  IntegratorStateMustResolveToSignalObject=off  IntegratorRTWStateStorageClass=Auto  FilterContinuousStateAttributes=''  FilterStateMustResolveToSignalObject=off  FilterRTWStateStorageClass=Auto  ParallelPVariant=ExternalParameters  IdealPVariant=Disabled  IVariant=ExternalParameters  DVariant=Disabled  IntegratorVariant=Discrete  SatVariant=Enabled  AWVariant=DiscClampingParallel  PCopyVariant=Disabled  TRVariant=Disabled  FdbkBlocksVariant=Forward  IdealPFdbkVariant=Disabled  SatFdbkVariant=Disabled  DerivativeFilterVariant=Disabled  NVariant=Disabled  NCopyVariant=Disabled_SignalSpec  FilterICVariant=Disabled  IntegratorICVariant=InternalICs  ExternalResetVariant=Disabled  TRSumVariant=Passthrough  SumFdbkVariant=Disabled  SumVariant=Sum_PI  TsampFilterVariant=InternalTs  TsampNgainVariant=Passthrough  TsampIntegralVariant=Passthrough  ExternalSaturationOutDataTypeStr=Inherit: Same as second input
  Saturation : Saturate  UpperLimit=30000  LowerLimit=-99999
  Sum4 : Sum  Inputs=|+-
  dT1 : Outport
  wires:
  i/1 -> PID Controller/3
  p/1 -> PID Controller/2
  PID Controller/1 -> Saturation/1  "dT1"
  lamda2/1 -> Sum4/2
  Sum4/1 -> PID Controller/1
  Saturation/1 -> dT1/1
  Constant/1 -> Sum4/1

== system tractor_mu/驱动防滑模块/Subsystem2 ==
  lamda3 : Inport
  p : Inport  Port=2
  i : Inport  Port=3
  b : Inport  Port=4
  Constant : Constant  Value=0.2
  PID Controller : slpidlib/PID Controller  Controller=PI  Form=Parallel  TimeDomain=Discrete-time  UseExternalTs=off  SampleTime=-1  IntegratorMethod=Forward Euler  FilterMethod=Forward Euler  ControllerParametersSource=external  P=5000  I=3000  UseKiTs=off  D=0  N=100  UseFilter=on  TunerSelectOption=Transfer Function Based (PID Tuner App)  InitialConditionSource=internal  InitialConditionForIntegrator=0  InitialConditionForFilter=0  DifferentiatorICPrevScaledInput=0  ExternalReset=none  TrackingMode=off  Kt=1  LimitOutput=on  SatLimitsSource=internal  UpperSaturationLimit=0  LowerSaturationLimit=-50000  LinearizeAsGain=on  AntiWindupMode=clamping  Kb=1  LimitIntegrator=off  UpperIntegratorSaturationLimit=inf  LowerIntegratorSaturationLimit=-inf  POutMin=[]  POutMax=[]  IOutMin=[]  IOutMax=[]  DOutMin=[]  DOutMax=[]  NOutMin=[]  NOutMax=[]  SumOutMin=[]  SumOutMax=[]  SaturationOutMin=[]  SaturationOutMax=[]  PParamMin=[]  PParamMax=[]  IParamMin=[]  IParamMax=[]  DParamMin=[]  DParamMax=[]  NParamMin=[]  NParamMax=[]  KbParamMin=[]  KbParamMax=[]  KtParamMin=[]  KtParamMax=[]  KbOutMin=[]  KbOutMax=[]  KtOutMin=[]  KtOutMax=[]  IntegratorOutMin=[]  IntegratorOutMax=[]  FilterOutMin=[]  FilterOutMax=[]  SumI1OutMin=[]  SumI1OutMax=[]  SumI2OutMin=[]  SumI2OutMax=[]  SumI3OutMin=[]  SumI3OutMax=[]  SumI4OutMin=[]  SumI4OutMax=[]  SumDOutMin=[]  SumDOutMax=[]  DifferentiatorOutMin=[]  DifferentiatorOutMax=[]  FilterDiffOutCoefMin=[]  FilterDiffOutCoefMax=[]  ReciprocalOutMin=[]  ReciprocalOutMax=[]  SumDenOutMin=[]  SumDenOutMax=[]  SumNumOutMin=[]  SumNumOutMax=[]  DivideOutMin=[]  DivideOutMax=[]  UdiffTsProdOutMin=[]  UdiffTsProdOutMax=[]  NTsProdOutMin=[]  NTsProdOutMax=[]  UintegralTsProdOutMin=[]  UintegralTsProdOutMax=[]  UngainTsProdOutMin=[]  UngainTsProdOutMax=[]  ClampingZeroOutDataTypeStr=Inherit: Inherit via back propagation  ClampingZeroOutMin=[]  ClampingZeroOutMax=[]  FilterDenConstantOutDataTypeStr=Inherit: Inherit via back propagation  FilterDenConstantOutMin=[]  FilterDenConstantOutMax=[]  PCopyOutDataTypeStr=Inherit: Inherit via back propagation  PCopyOutMin=[]  PCopyOutMax=[]  NCopyOutDataTypeStr=Inherit: Inherit via back propagation  NCopyOutMin=[]  NCopyOutMax=[]  IntegratorContinuousStateAttributes=''  IntegratorStateMustResolveToSignalObject=off  IntegratorRTWStateStorageClass=Auto  FilterContinuousStateAttributes=''  FilterStateMustResolveToSignalObject=off  FilterRTWStateStorageClass=Auto  ParallelPVariant=ExternalParameters  IdealPVariant=Disabled  IVariant=ExternalParameters  DVariant=Disabled  IntegratorVariant=Discrete  SatVariant=Enabled  AWVariant=DiscClampingParallel  PCopyVariant=Disabled  TRVariant=Disabled  FdbkBlocksVariant=Forward  IdealPFdbkVariant=Disabled  SatFdbkVariant=Disabled  DerivativeFilterVariant=Disabled  NVariant=Disabled  NCopyVariant=Disabled_SignalSpec  FilterICVariant=Disabled  IntegratorICVariant=InternalICs  ExternalResetVariant=Disabled  TRSumVariant=Passthrough  SumFdbkVariant=Disabled  SumVariant=Sum_PI  TsampFilterVariant=InternalTs  TsampNgainVariant=Passthrough  TsampIntegralVariant=Passthrough  ExternalSaturationOutDataTypeStr=Inherit: Same as second input
  Saturation : Saturate  UpperLimit=30000  LowerLimit=-99999
  Sum4 : Sum  Inputs=|+-
  dT1 : Outport
  wires:
  Sum4/1 -> PID Controller/1
  lamda3/1 -> Sum4/2
  PID Controller/1 -> Saturation/1  "dT1"
  p/1 -> PID Controller/2
  i/1 -> PID Controller/3
  Saturation/1 -> dT1/1
  Constant/1 -> Sum4/1

== system tractor_mu/驱动防滑模块/Subsystem3 ==
  lamda4 : Inport
  p : Inport  Port=2
  i : Inport  Port=3
  b : Inport  Port=4
  Constant : Constant  Value=0.2
  PID Controller : slpidlib/PID Controller  Controller=PI  Form=Parallel  TimeDomain=Discrete-time  UseExternalTs=off  SampleTime=-1  IntegratorMethod=Forward Euler  FilterMethod=Forward Euler  ControllerParametersSource=external  P=5000  I=3000  UseKiTs=off  D=0  N=100  UseFilter=on  TunerSelectOption=Transfer Function Based (PID Tuner App)  InitialConditionSource=internal  InitialConditionForIntegrator=0  InitialConditionForFilter=0  DifferentiatorICPrevScaledInput=0  ExternalReset=none  TrackingMode=off  Kt=1  LimitOutput=on  SatLimitsSource=internal  UpperSaturationLimit=0  LowerSaturationLimit=-50000  LinearizeAsGain=on  AntiWindupMode=clamping  Kb=1  LimitIntegrator=off  UpperIntegratorSaturationLimit=inf  LowerIntegratorSaturationLimit=-inf  POutMin=[]  POutMax=[]  IOutMin=[]  IOutMax=[]  DOutMin=[]  DOutMax=[]  NOutMin=[]  NOutMax=[]  SumOutMin=[]  SumOutMax=[]  SaturationOutMin=[]  SaturationOutMax=[]  PParamMin=[]  PParamMax=[]  IParamMin=[]  IParamMax=[]  DParamMin=[]  DParamMax=[]  NParamMin=[]  NParamMax=[]  KbParamMin=[]  KbParamMax=[]  KtParamMin=[]  KtParamMax=[]  KbOutMin=[]  KbOutMax=[]  KtOutMin=[]  KtOutMax=[]  IntegratorOutMin=[]  IntegratorOutMax=[]  FilterOutMin=[]  FilterOutMax=[]  SumI1OutMin=[]  SumI1OutMax=[]  SumI2OutMin=[]  SumI2OutMax=[]  SumI3OutMin=[]  SumI3OutMax=[]  SumI4OutMin=[]  SumI4OutMax=[]  SumDOutMin=[]  SumDOutMax=[]  DifferentiatorOutMin=[]  DifferentiatorOutMax=[]  FilterDiffOutCoefMin=[]  FilterDiffOutCoefMax=[]  ReciprocalOutMin=[]  ReciprocalOutMax=[]  SumDenOutMin=[]  SumDenOutMax=[]  SumNumOutMin=[]  SumNumOutMax=[]  DivideOutMin=[]  DivideOutMax=[]  UdiffTsProdOutMin=[]  UdiffTsProdOutMax=[]  NTsProdOutMin=[]  NTsProdOutMax=[]  UintegralTsProdOutMin=[]  UintegralTsProdOutMax=[]  UngainTsProdOutMin=[]  UngainTsProdOutMax=[]  ClampingZeroOutDataTypeStr=Inherit: Inherit via back propagation  ClampingZeroOutMin=[]  ClampingZeroOutMax=[]  FilterDenConstantOutDataTypeStr=Inherit: Inherit via back propagation  FilterDenConstantOutMin=[]  FilterDenConstantOutMax=[]  PCopyOutDataTypeStr=Inherit: Inherit via back propagation  PCopyOutMin=[]  PCopyOutMax=[]  NCopyOutDataTypeStr=Inherit: Inherit via back propagation  NCopyOutMin=[]  NCopyOutMax=[]  IntegratorContinuousStateAttributes=''  IntegratorStateMustResolveToSignalObject=off  IntegratorRTWStateStorageClass=Auto  FilterContinuousStateAttributes=''  FilterStateMustResolveToSignalObject=off  FilterRTWStateStorageClass=Auto  ParallelPVariant=ExternalParameters  IdealPVariant=Disabled  IVariant=ExternalParameters  DVariant=Disabled  IntegratorVariant=Discrete  SatVariant=Enabled  AWVariant=DiscClampingParallel  PCopyVariant=Disabled  TRVariant=Disabled  FdbkBlocksVariant=Forward  IdealPFdbkVariant=Disabled  SatFdbkVariant=Disabled  DerivativeFilterVariant=Disabled  NVariant=Disabled  NCopyVariant=Disabled_SignalSpec  FilterICVariant=Disabled  IntegratorICVariant=InternalICs  ExternalResetVariant=Disabled  TRSumVariant=Passthrough  SumFdbkVariant=Disabled  SumVariant=Sum_PI  TsampFilterVariant=InternalTs  TsampNgainVariant=Passthrough  TsampIntegralVariant=Passthrough  ExternalSaturationOutDataTypeStr=Inherit: Same as second input
  Saturation : Saturate  UpperLimit=30000  LowerLimit=-99999
  Sum4 : Sum  Inputs=|+-
  dT1 : Outport
  wires:
  i/1 -> PID Controller/3
  p/1 -> PID Controller/2
  PID Controller/1 -> Saturation/1  "dT1"
  lamda4/1 -> Sum4/2
  Sum4/1 -> PID Controller/1
  Saturation/1 -> dT1/1
  Constant/1 -> Sum4/1

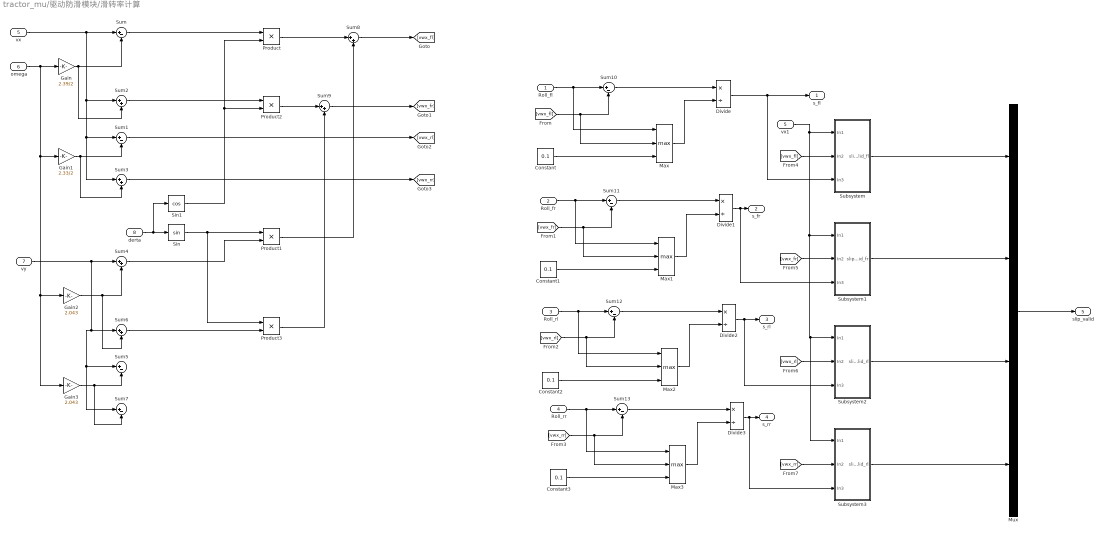
== system tractor_mu/驱动防滑模块/滑转率计算 ==
  Roll_fl : Inport
  Roll_fr : Inport  Port=2
  Roll_rl : Inport  Port=3
  Roll_rr : Inport  Port=4
  vx : Inport  Port=5
  omega : Inport  Port=6
  vy : Inport  Port=7
  derta : Inport  Port=8
  Constant{,1..3} (4 alike) : Constant  Value=0.1
  Divide{,1..3} (4 alike) : Product  Inputs=*/
  Gain : Gain  Gain=2.39/2
  Gain1 : Gain  Gain=2.33/2
  Gain2 : Gain  Gain=2.043
  Gain3 : Gain  Gain=2.043
  Max{,1..3} (4 alike) : MinMax  Function=max  Inputs=3
  Mux : Mux
  Product{,1..3} (4 alike) : Product
  Sin : Trigonometry
  Sin1 : Trigonometry  Operator=cos
  Subsystem : Subsystem
  Subsystem1 : Subsystem
  Subsystem2 : Subsystem
  Subsystem3 : Subsystem
  Sum{,1,5,7,10..13} (8 alike) : Sum  Inputs=|+-
  Sum{2..4,6,8..9} (6 alike) : Sum  Inputs=|++
  vx1 : InportShadow  Port=5
  s_fl : Outport
  s_fr : Outport  Port=2
  s_rl : Outport  Port=3
  s_rr : Outport  Port=4
  slip_valid : Outport  Port=5
  wires:
  vx/1 -> Sum3/1, Sum1/1, Sum2/1, Sum/1
  Gain/1 -> Sum2/2, Sum/2
  Gain1/1 -> Sum3/2, Sum1/2
  Gain3/1 -> Sum5/2, Sum7/2
  Gain2/1 -> Sum4/2, Sum6/2
  omega/1 -> Gain3/1, Gain2/1, Gain1/1, Gain/1
  vy/1 -> Sum4/1, Sum5/1, Sum7/1, Sum6/1
  derta/1 -> Sin1/1, Sin/1
  Sum/1 -> Product/1
  Sin1/1 -> Product2/2, Product/2
  Product/1 -> Sum8/1
  Sin/1 -> Product3/1, Product1/1
  Sum4/1 -> Product1/2
  Product1/1 -> Sum8/2
  Sum8/1 -> [vwx_fl]
  Sum2/1 -> Product2/1
  Product2/1 -> Sum9/1
  Sum6/1 -> Product3/2
  Product3/1 -> Sum9/2
  Sum9/1 -> [vwx_fr]
  Sum1/1 -> [vwx_rl]
  Sum3/1 -> [vwx_rr]
  Roll_fl/1 -> Max/1, Sum10/1
  [vwx_fl] -> Max/2, Sum10/2
  Sum10/1 -> Divide/1
  Constant/1 -> Max/3
  Max/1 -> Divide/2
  Divide/1 -> Subsystem/3(In3), s_fl/1
  Divide1/1 -> Subsystem1/3(In3), s_fr/1
  Max1/1 -> Divide1/2
  Constant1/1 -> Max1/3
  Sum11/1 -> Divide1/1
  [vwx_fr] -> Sum11/2, Max1/2
  Roll_fr/1 -> Sum11/1, Max1/1
  Roll_rl/1 -> Max2/1, Sum12/1
  [vwx_rl] -> Max2/2, Sum12/2
  Sum12/1 -> Divide2/1
  Constant2/1 -> Max2/3
  Max2/1 -> Divide2/2
  Divide2/1 -> Subsystem2/3(In3), s_rl/1
  Divide3/1 -> Subsystem3/3(In3), s_rr/1
  Max3/1 -> Divide3/2
  Constant3/1 -> Max3/3
  Sum13/1 -> Divide3/1
  [vwx_rr] -> Sum13/2, Max3/2
  Roll_rr/1 -> Sum13/1, Max3/1
  vx1/1 -> Subsystem3/1(In1), Subsystem2/1(In1), Subsystem1/1(In1), Subsystem/1(In1)
  [vwx_fl] -> Subsystem/2(In2)
  [vwx_fr] -> Subsystem1/2(In2)
  [vwx_rl] -> Subsystem2/2(In2)
  [vwx_rr] -> Subsystem3/2(In2)
  Subsystem/1(slip_valid_fl) -> Mux/1
  Subsystem1/1(slip_valid_fr) -> Mux/2
  Subsystem2/1(slip_valid_rl) -> Mux/3
  Subsystem3/1(slip_valid_rl) -> Mux/4
  Mux/1 -> slip_valid/1

== system tractor_mu/Dugoff轮胎模型/alpha_lamda/alpha ==
  vx : Inport
  vy : Inport  Port=2
  wz : Inport  Port=3
  delta_fl : Inport  Port=4
  delta_fr : Inport  Port=5
  Gain{,1..3} (4 alike) : Gain  Gain=-1
  fl : Subsystem
  fr : Subsystem
  rl : Subsystem
  rr : Subsystem
  alpha_fl : Outport
  alpha_fr : Outport  Port=2
  alpha_rl : Outport  Port=3
  alpha_rr : Outport  Port=4
  wires:
  delta_fr/1 -> fr/4(delta_fr)
  delta_fl/1 -> fl/4(delta_fl)
  vy/1 -> rl/2(vy), fl/2(vy), fr/2(vy), rr/2(vy)
  vx/1 -> rl/1(vx), fl/1(vx), fr/1(vx), rr/1(vx)
  wz/1 -> rl/3(wz), fr/3(wz), rr/3(wz), fl/3(wz)
  fl/1(alpha_fl) -> Gain/1
  Gain/1 -> alpha_fl/1
  rl/1(alpha_rl) -> Gain1/1
  Gain1/1 -> alpha_rl/1
  fr/1(alpha_fr) -> Gain2/1
  Gain2/1 -> alpha_fr/1
  rr/1(alpha_rr) -> Gain3/1
  Gain3/1 -> alpha_rr/1

== system tractor_mu/Dugoff轮胎模型/alpha_lamda/lamda ==
  vx : Inport
  vy : Inport  Port=2
  wz : Inport  Port=3
  delta_fl : Inport  Port=4
  delta_fr : Inport  Port=5
  w_fl : Inport  Port=6
  w_fr : Inport  Port=7
  w_rl : Inport  Port=8
  w_rr : Inport  Port=9
  fl : Subsystem
  fr : Subsystem
  rl : Subsystem
  rr : Subsystem
  lamda_fl : Outport
  lamda_fr : Outport  Port=2
  lamda_rl : Outport  Port=3
  lamda_rr : Outport  Port=4
  wires:
  fr/1(lamda_fr) -> lamda_fr/1
  rr/1(lamda_rr) -> lamda_rr/1
  w_rl/1 -> rl/1(w_rl)
  w_rr/1 -> rr/1(w_rr)
  w_fr/1 -> fr/1(w_fr)
  delta_fr/1 -> fr/5(delta_fr)
  delta_fl/1 -> fl/5(delta_fl)
  vy/1 -> fl/4(vy), fr/4(vy)
  vx/1 -> fl/3(vx), fr/3(vx), rr/3(vx), rl/3(vx)
  wz/1 -> fl/2(wz), fr/2(wz), rr/2(wz), rl/2(wz)
  w_fl/1 -> fl/1(w_fl)
  rl/1(lamda_rl) -> lamda_rl/1
  fl/1(lamda_fl) -> lamda_fl/1

== system tractor_mu/四轮转矩分配/下层轮胎力执行控制器/右前轮 ==
  FzR1 : Inport
  FxR1 : Inport  Port=2
  FyR1 : Inport  Port=3
  kappa_R1 : Inport  Port=4
  derta : Inport  Port=5
  Gain : Gain  Gain=0.834
  If : If  IfExpression=u1 > 52000  ElseIfExpressions=u1<18000
  If Action Subsystem : Subsystem  TreatAsAtomicUnit=on
  If Action Subsystem1 : Subsystem  TreatAsAtomicUnit=on
  If Action Subsystem2 : Subsystem  TreatAsAtomicUnit=on
  Merge : Merge  Inputs=3
  PID Controller : slpidlib/PID Controller  Controller=PID  Form=Parallel  TimeDomain=Discrete-time  UseExternalTs=off  SampleTime=-1  IntegratorMethod=Forward Euler  FilterMethod=Forward Euler  ControllerParametersSource=internal  P=3500  I=3000  UseKiTs=off  D=0  N=100  UseFilter=on  TunerSelectOption=Transfer Function Based (PID Tuner App)  InitialConditionSource=internal  InitialConditionForIntegrator=0  InitialConditionForFilter=0  DifferentiatorICPrevScaledInput=0  ExternalReset=none  TrackingMode=off  Kt=1  LimitOutput=off  SatLimitsSource=internal  UpperSaturationLimit=inf  LowerSaturationLimit=-inf  LinearizeAsGain=on  AntiWindupMode=none  Kb=1  LimitIntegrator=off  UpperIntegratorSaturationLimit=inf  LowerIntegratorSaturationLimit=-inf  POutMin=[]  POutMax=[]  IOutMin=[]  IOutMax=[]  DOutMin=[]  DOutMax=[]  NOutMin=[]  NOutMax=[]  SumOutMin=[]  SumOutMax=[]  SaturationOutMin=[]  SaturationOutMax=[]  PParamMin=[]  PParamMax=[]  IParamMin=[]  IParamMax=[]  DParamMin=[]  DParamMax=[]  NParamMin=[]  NParamMax=[]  KbParamMin=[]  KbParamMax=[]  KtParamMin=[]  KtParamMax=[]  KbOutMin=[]  KbOutMax=[]  KtOutMin=[]  KtOutMax=[]  IntegratorOutMin=[]  IntegratorOutMax=[]  FilterOutMin=[]  FilterOutMax=[]  SumI1OutMin=[]  SumI1OutMax=[]  SumI2OutMin=[]  SumI2OutMax=[]  SumI3OutMin=[]  SumI3OutMax=[]  SumI4OutMin=[]  SumI4OutMax=[]  SumDOutMin=[]  SumDOutMax=[]  DifferentiatorOutMin=[]  DifferentiatorOutMax=[]  FilterDiffOutCoefMin=[]  FilterDiffOutCoefMax=[]  ReciprocalOutMin=[]  ReciprocalOutMax=[]  SumDenOutMin=[]  SumDenOutMax=[]  SumNumOutMin=[]  SumNumOutMax=[]  DivideOutMin=[]  DivideOutMax=[]  UdiffTsProdOutMin=[]  UdiffTsProdOutMax=[]  NTsProdOutMin=[]  NTsProdOutMax=[]  UintegralTsProdOutMin=[]  UintegralTsProdOutMax=[]  UngainTsProdOutMin=[]  UngainTsProdOutMax=[]  ClampingZeroOutDataTypeStr=Inherit: Inherit via back propagation  ClampingZeroOutMin=[]  ClampingZeroOutMax=[]  FilterDenConstantOutDataTypeStr=Inherit: Inherit via back propagation  FilterDenConstantOutMin=[]  FilterDenConstantOutMax=[]  PCopyOutDataTypeStr=Inherit: Inherit via back propagation  PCopyOutMin=[]  PCopyOutMax=[]  NCopyOutDataTypeStr=Inherit: Inherit via back propagation  NCopyOutMin=[]  NCopyOutMax=[]  IntegratorContinuousStateAttributes=''  IntegratorStateMustResolveToSignalObject=off  IntegratorRTWStateStorageClass=Auto  FilterContinuousStateAttributes=''  FilterStateMustResolveToSignalObject=off  FilterRTWStateStorageClass=Auto  ParallelPVariant=InternalParameters  IdealPVariant=Disabled  IVariant=InternalParameters  DVariant=InternalParameters  IntegratorVariant=Discrete  SatVariant=Disabled  AWVariant=Passthrough  PCopyVariant=Disabled  TRVariant=Disabled  FdbkBlocksVariant=Forward  IdealPFdbkVariant=Disabled  SatFdbkVariant=Disabled  DerivativeFilterVariant=ForwardEulerFilter  NVariant=InternalParameters  NCopyVariant=Disabled  FilterICVariant=InternalICsFilter  IntegratorICVariant=InternalICs  ExternalResetVariant=Disabled  TRSumVariant=Passthrough  SumFdbkVariant=Disabled  SumVariant=Sum_PID  TsampFilterVariant=InternalTs  TsampNgainVariant=Passthrough  TsampIntegralVariant=Passthrough  ExternalSaturationOutDataTypeStr=Inherit: Same as second input
  Product : Product
  Product1 : Product
  Saturation1 : Saturate  UpperLimit=1100*63.52  LowerLimit=0
  Sin : Trigonometry
  Sin1 : Trigonometry  Operator=cos
  Sum : Sum  Inputs=|++
  Sum1 : Sum  Inputs=|+-
  Sum2 : Sum  Inputs=|++
  Torque2 : Scope  NumInputPorts=2
  kappa2 : Scope  NumInputPorts=2
  Out1 : Outport
  wires:
  If Action Subsystem1/1(kappa_d) -> Merge/1
  If Action Subsystem2/1(kappa_d) -> Merge/3
  Product1/1 -> Sum/1
  Gain/1 -> Sum2/2
  Product/1 -> Sum/2
  Sin1/1 -> Product1/2
  If/3 -> If Action Subsystem2/Action
  derta/1 -> Sin/1, Sin1/1
  Sum/1 -> Gain/1
  kappa_R1/1 -> kappa2/2, Sum1/2
  FzR1/1 -> If/1
  If Action Subsystem/1(kappa_d) -> Merge/2
  If/2 -> If Action Subsystem/Action
  FyR1/1 -> Product/1
  Sum2/1 -> Torque2/2, Saturation1/1
  Sin/1 -> Product/2
  FxR1/1 -> If Action Subsystem/1(Fx), If Action Subsystem1/1(Fx), If Action Subsystem2/1(Fx), Product1/1
  If/1 -> If Action Subsystem1/Action
  Saturation1/1 -> Out1/1
  Sum1/1 -> PID Controller/1
  Merge/1 -> kappa2/1, Sum1/1
  PID Controller/1 -> Torque2/1, Sum2/1
